simulink model "Three_blocks_continuous"  (R2017b)
settings: Solver=VariableStepAuto  StartTime=0.0  StopTime=100  RelTol=1e-3
libraries: simulink x3
settings Model: Creator=giuli  LastModifiedBy=giuli

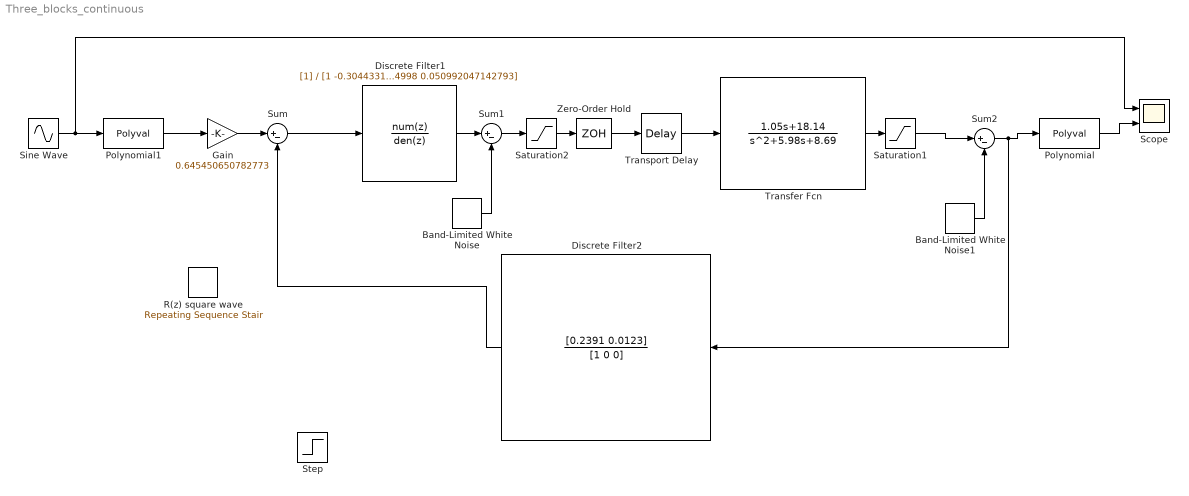
== system Three_blocks_continuous ==
  Band-Limited White Noise : simulink/Sources/Band-Limited White Noise  Cov=[0.01]  Ts=0.08  seed=[23341]
  Band-Limited White Noise1 : simulink/Sources/Band-Limited White Noise  Cov=[0.01]  Ts=0.08  seed=[23341]
  Discrete Filter1 : DiscreteFilter  Denominator=[1 -0.304433146028352 0.094556540964998 0.050992047142793]  SampleTime=0.08
  Discrete Filter2 : DiscreteFilter  Numerator=[0.2391 0.0123]  Denominator=[1 0 0]  SampleTime=0.08
  Gain : Gain  Gain=0.645450650782773
  Polynomial : Polyval  Coefs=[2.865 26.323]
  Polynomial1 : Polyval  Coefs=[1/2.865 -26.323/2.865]
  R(z) square wave : simulink/Sources/Repeating Sequence Stair  OutValues=[15 45 40 30 25 30 40]  tsamp=20  OutMin=[]  OutMax=[]  OutDataTypeStr=double  OutputDataTypeScalingMode=double  OutDataType=fixdt(0,8)  ConRadixGroup=Best Precision: Vector-wise  OutScaling=2^-12
  Saturation1 : Saturate  UpperLimit=10  LowerLimit=-10
  Saturation2 : Saturate  UpperLimit=5  LowerLimit=0
  Scope : Scope  NumInputPorts=2
  Sine Wave : Sin  Amplitude=10  Bias=35  Frequency=0.1  SampleTime=0
  Step : Step  Before=15  After=55  SampleTime=0.08
  Sum : Sum  Inputs=|+-
  Sum1 : Sum  Inputs=|+-
  Sum2 : Sum  Inputs=|+-
  Transfer Fcn : TransferFcn  Numerator=[1.05 18.14]  Denominator=[1 5.98 8.69]
  Transport Delay : TransportDelay  DelayTime=0.2
  Zero-Order Hold : ZeroOrderHold  SampleTime=-1
  wires:
  Sum/1 -> Discrete Filter1/1
  Sine Wave/1 -> Polynomial1/1, Scope/1
  Gain/1 -> Sum/1
  Polynomial1/1 -> Gain/1
  Discrete Filter2/1 -> Sum/2
  Zero-Order Hold/1 -> Transport Delay/1
  Transport Delay/1 -> Transfer Fcn/1
  Transfer Fcn/1 -> Saturation1/1
  Saturation2/1 -> Zero-Order Hold/1
  Discrete Filter1/1 -> Sum1/1
  Band-Limited White Noise/1 -> Sum1/2
  Sum1/1 -> Saturation2/1
  Band-Limited White Noise1/1 -> Sum2/2
  Saturation1/1 -> Sum2/1
  Sum2/1 -> Discrete Filter2/1, Polynomial/1
  Polynomial/1 -> Scope/2
